simulink model "fw_safety_supervisor"  (R2026b)
settings: Solver=VariableStepAuto
undefined symbols (not defined in the file or in its folder): ImplementType, P, ShaddadMode, Ts
libraries: simulink x65
settings Model: Creator=aomar  LastModifiedBy=aomar

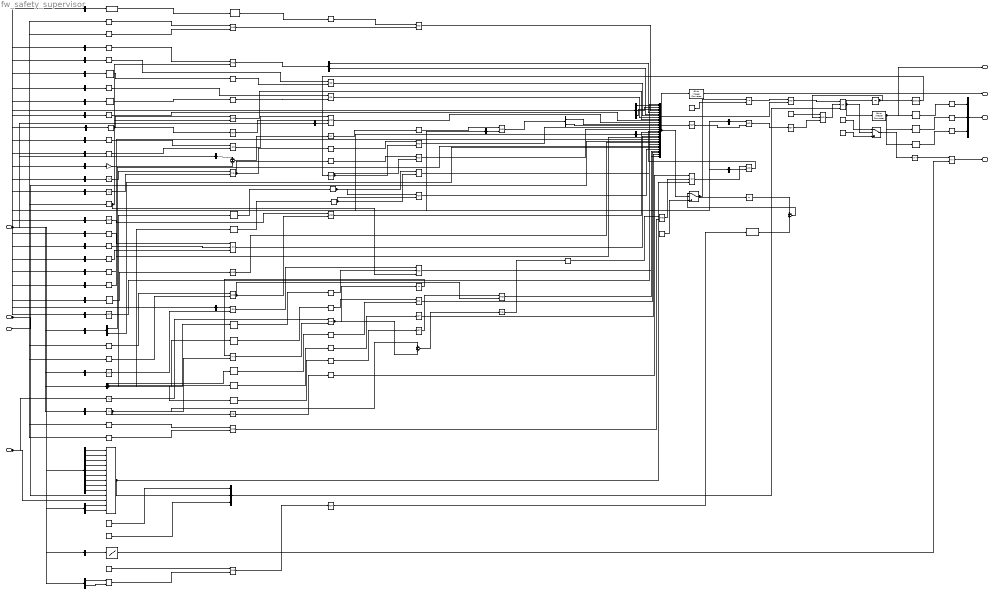
== system fw_safety_supervisor ==
  fw10 : Inport  SampleTime=Ts.ctrl
  mode_prev : Inport  Port=2  OutDataTypeStr=uint8  SampleTime=Ts.ctrl
  stop_fail_prev : Inport  Port=3  OutDataTypeStr=boolean  SampleTime=Ts.ctrl
  vtrack_ref_prev : Inport  Port=4  OutDataTypeStr=single  PortDimensions=2  SampleTime=Ts.ctrl
  Act : Logic  AllPortsSameDT=off  OutDataTypeStr=boolean
  Act_hi : simulink/Logic and Bit Operations/Compare To Constant  relop=<=  const=double(ShaddadMode.CTRL_STOP)  OutDataTypeStr=boolean
  Act_lo : simulink/Logic and Bit Operations/Compare To Constant  relop=>=  const=double(ShaddadMode.MANUAL)  OutDataTypeStr=boolean
  Active : Logic  Operator=OR  Inputs=3  AllPortsSameDT=off  OutDataTypeStr=boolean
  Auto : Logic  AllPortsSameDT=off  OutDataTypeStr=boolean
  Auto_hi : simulink/Logic and Bit Operations/Compare To Constant  relop=<=  const=double(ShaddadMode.AUTO)  OutDataTypeStr=boolean
  Auto_lo : simulink/Logic and Bit Operations/Compare To Constant  relop=>=  const=double(ShaddadMode.AUTO_START)  OutDataTypeStr=boolean
  Bms_dcl_low : simulink/Logic and Bit Operations/Compare To Constant  relop=<  const=P.electronics.safety.dcl_warn  OutDataTypeStr=boolean
  Bms_fresh : Logic  Operator=NOT  Inputs=1  AllPortsSameDT=off  OutDataTypeStr=boolean
  Bms_stale : simulink/Logic and Bit Operations/Compare To Constant  relop=>  const=P.electronics.safety.bms_timeout + Ts.hk/2  OutDataTypeStr=boolean
  Bms_warn_any : Logic  Operator=OR  AllPortsSameDT=off  OutDataTypeStr=boolean
  Bms_warnword : simulink/Logic and Bit Operations/Compare To Zero  relop=~=  OutDataTypeStr=boolean
  Busoff : Demux  Outputs=2
  C00_hw_estop : Logic  Operator=NAND  AllPortsSameDT=off  OutDataTypeStr=boolean
  C04_comp_timeout : Logic  AllPortsSameDT=off  OutDataTypeStr=boolean
  C07_drv_fault_L : Logic  Operator=OR  AllPortsSameDT=off  OutDataTypeStr=boolean
  C08_drv_fault_R : Logic  Operator=OR  AllPortsSameDT=off  OutDataTypeStr=boolean
  C09_bms_timeout : Logic  AllPortsSameDT=off  OutDataTypeStr=boolean
  C10_bms_alarm : simulink/Logic and Bit Operations/Compare To Constant  relop===  const=3  OutDataTypeStr=boolean
  C11_bms_warn : Logic  Inputs=3  AllPortsSameDT=off  OutDataTypeStr=boolean
  C14_tilt_warn : Logic  AllPortsSameDT=off  OutDataTypeStr=boolean
  C15_tilt_stop : Logic  AllPortsSameDT=off  OutDataTypeStr=boolean
  C16_overspeed : Logic  AllPortsSameDT=off  OutDataTypeStr=boolean
  C17_hv_lost : Logic  AllPortsSameDT=off  OutDataTypeStr=boolean
  C19_rail_uv : Logic  Operator=OR  Inputs=3  AllPortsSameDT=off  OutDataTypeStr=boolean
  C20_encl_warn : simulink/Logic and Bit Operations/Compare To Constant  relop=>  const=P.electronics.safety.T_encl_warn  OutDataTypeStr=boolean
  C21_encl_crit : simulink/Logic and Bit Operations/Compare To Constant  relop=>  const=P.electronics.safety.T_encl_crit  OutDataTypeStr=boolean
  C23_overrun : Logic  Inputs=1  AllPortsSameDT=off  OutDataTypeStr=boolean
  C24_imu_fault : Logic  Operator=NOT  Inputs=1  AllPortsSameDT=off  OutDataTypeStr=boolean
  C27_discrepancy : Logic  Operator=XOR  AllPortsSameDT=off  OutDataTypeStr=boolean
  C28_impl_fault : Logic  Inputs=3  AllPortsSameDT=off  OutDataTypeStr=boolean
  C29_bumper : Logic  Operator=OR  AllPortsSameDT=off  OutDataTypeStr=boolean
  C30_lid_open : Logic  Operator=NOT  Inputs=1  AllPortsSameDT=off  OutDataTypeStr=boolean
  C31_relay_open : Logic  AllPortsSameDT=off  OutDataTypeStr=boolean
  Clear : Logic  AllPortsSameDT=off  OutDataTypeStr=boolean
  Cls : Concatenate  NumInputs=3
  Cls_A : simulink/Logic and Bit Operations/Compare To Zero  relop=~=  OutDataTypeStr=boolean
  Cls_A_mask : simulink/Logic and Bit Operations/Bitwise Operator  logicop=AND  UseBitMask=on  BitMask=P.electronics.safety.maskA  BitMaskRealWorld=Stored Integer
  Cls_B : simulink/Logic and Bit Operations/Compare To Zero  relop=~=  OutDataTypeStr=boolean
  Cls_B_mask : simulink/Logic and Bit Operations/Bitwise Operator  logicop=AND  UseBitMask=on  BitMask=P.electronics.safety.maskB  BitMaskRealWorld=Stored Integer
  Cls_C : simulink/Logic and Bit Operations/Compare To Zero  relop=~=  OutDataTypeStr=boolean
  Cls_C_mask : simulink/Logic and Bit Operations/Bitwise Operator  logicop=AND  UseBitMask=on  BitMask=P.electronics.safety.maskC  BitMaskRealWorld=Stored Integer
  Cnt : Switch  Criteria=u2 ~= 0  SaturateOnIntegerOverflow=off  InputSameDT=off
  Cnt_inc : Sum  OutDataTypeStr=uint16  SaturateOnIntegerOverflow=on
  Cnt_prev : UnitDelay  InitialCondition=zeros(1,32)  SampleTime=-1
  Cnt_zero : Constant  Value=zeros(1,32)  OutDataTypeStr=uint16  SampleTime=Ts.ctrl
  Cond : Concatenate  NumInputs=32
  Cond_not : Logic  Operator=NOT  Inputs=1  AllPortsSameDT=off  OutDataTypeStr=boolean
  Count_tick : Logic  Operator=NOT  Inputs=1  AllPortsSameDT=off  OutDataTypeStr=boolean
  DI_bumper_front : simulink/Logic and Bit Operations/Compare To Zero  relop=~=  OutDataTypeStr=boolean
  DI_bumper_front_mask : simulink/Logic and Bit Operations/Bitwise Operator  logicop=AND  UseBitMask=on  BitMask=2^(P.electronics.di.bumper_front)  BitMaskRealWorld=Stored Integer
  DI_bumper_rear : simulink/Logic and Bit Operations/Compare To Zero  relop=~=  OutDataTypeStr=boolean
  DI_bumper_rear_mask : simulink/Logic and Bit Operations/Bitwise Operator  logicop=AND  UseBitMask=on  BitMask=2^(P.electronics.di.bumper_rear)  BitMaskRealWorld=Stored Integer
  DI_estop_ch1_ok : simulink/Logic and Bit Operations/Compare To Zero  relop=~=  OutDataTypeStr=boolean
  DI_estop_ch1_ok_mask : simulink/Logic and Bit Operations/Bitwise Operator  logicop=AND  UseBitMask=on  BitMask=2^(P.electronics.di.estop_ch1_ok)  BitMaskRealWorld=Stored Integer
  DI_estop_ch2_ok : simulink/Logic and Bit Operations/Compare To Zero  relop=~=  OutDataTypeStr=boolean
  DI_estop_ch2_ok_mask : simulink/Logic and Bit Operations/Bitwise Operator  logicop=AND  UseBitMask=on  BitMask=2^(P.electronics.di.estop_ch2_ok)  BitMaskRealWorld=Stored Integer
  DI_lid_closed : simulink/Logic and Bit Operations/Compare To Zero  relop=~=  OutDataTypeStr=boolean
  DI_lid_closed_mask : simulink/Logic and Bit Operations/Bitwise Operator  logicop=AND  UseBitMask=on  BitMask=2^(P.electronics.di.lid_closed)  BitMaskRealWorld=Stored Integer
  DI_safety_ok : simulink/Logic and Bit Operations/Compare To Zero  relop=~=  OutDataTypeStr=boolean
  DI_safety_ok_mask : simulink/Logic and Bit Operations/Bitwise Operator  logicop=AND  UseBitMask=on  BitMask=2^(P.electronics.di.safety_ok)  BitMaskRealWorld=Stored Integer
  Derate_bits : MinMax
  Derate_one : Constant  Value=ones(1,32)  OutDataTypeStr=single  SampleTime=Ts.ctrl
  Derate_sel : Switch  Criteria=u2 ~= 0  SaturateOnIntegerOverflow=off  InputSameDT=off
  Derate_therm : Lookup_n-D  NumberOfTableDimensions=1  BreakpointsForDimension1=P.electronics.aux.derate_bp  BreakpointsForDimension1DataTypeStr=single  Table=P.electronics.aux.derate_k  TableDataTypeStr=single  ExtrapMethod=Clip  InternalRulePriority=Speed  OutDataTypeStr=single  RndMeth=Simplest
  Derate_vec : Constant  Value=P.electronics.safety.derate_vec  OutDataTypeStr=single  SampleTime=Ts.ctrl
  Descent_trip : Subsystem
  Drv_old : simulink/Logic and Bit Operations/Compare To Constant  relop=>  const=P.electronics.safety.drv_timeout + Ts.ctrl/2  OutDataTypeStr=boolean
  Drv_on : Logic  AllPortsSameDT=off  OutDataTypeStr=boolean
  Drv_on_hi : simulink/Logic and Bit Operations/Compare To Constant  relop=<=  const=double(ShaddadMode.AUTO)  OutDataTypeStr=boolean
  Drv_on_lo : simulink/Logic and Bit Operations/Compare To Constant  relop=>=  const=double(ShaddadMode.MANUAL)  OutDataTypeStr=boolean
  Drv_tmo : Logic  AllPortsSameDT=off  OutDataTypeStr=boolean
  Drv_tmo_LR : Demux  Outputs=2
  Enc_abs : Abs  SaturateOnIntegerOverflow=off
  Enc_bad : simulink/Logic and Bit Operations/Compare To Constant  relop=>  const=P.electronics.drv.enc_mismatch_v  OutDataTypeStr=boolean
  Enc_diff : Sum  Inputs=+-
  Enc_mis : Logic  AllPortsSameDT=off  OutDataTypeStr=boolean
  Enc_mis_LR : Demux  Outputs=2
  Esc_fault_L : simulink/Logic and Bit Operations/Compare To Constant  relop===  const=P.electronics.safety.esc_fault_state  OutDataTypeStr=boolean
  Esc_fault_R : simulink/Logic and Bit Operations/Compare To Constant  relop===  const=P.electronics.safety.esc_fault_state  OutDataTypeStr=boolean
  Fault_pack : simulink/Logic and Bit Operations/Bit to Integer Converter  nbits=32  bitOrder=LSB first  signedOutputValues=Unsigned  outDtype=uint32  outDtypeSigned=Inherit via internal rule
      settings: LibrarySourceBlock=|
      | commutil2/Bit to Integer
      | Converter
  Fc_mask_L : simulink/Logic and Bit Operations/Bitwise Operator  logicop=AND  UseBitMask=on  BitMask=P.electronics.safety.drv_fault_mask  BitMaskRealWorld=Stored Integer
  Fc_mask_R : simulink/Logic and Bit Operations/Bitwise Operator  logicop=AND  UseBitMask=on  BitMask=P.electronics.safety.drv_fault_mask  BitMaskRealWorld=Stored Integer
  Fc_on_L : simulink/Logic and Bit Operations/Compare To Zero  relop=~=  OutDataTypeStr=boolean
  Fc_on_R : simulink/Logic and Bit Operations/Compare To Zero  relop=~=  OutDataTypeStr=boolean
  Follow_err : Sum  Inputs=+-
  Follow_max : MinMax  Function=max
  Follow_on : Logic  AllPortsSameDT=off  OutDataTypeStr=boolean
  Follow_over : simulink/Logic and Bit Operations/Compare To Constant  relop=>  const=P.electronics.lim.v_follow_dv  OutDataTypeStr=boolean
  Gate_bits : Constant  Value=bitget(sum(2.^[14 15]), 1:32) ~= 0  OutDataTypeStr=boolean  SampleTime=Ts.ctrl
  Gate_closed : Logic  Operator=NAND  AllPortsSameDT=off  OutDataTypeStr=boolean
  Held : Logic  Inputs=3  AllPortsSameDT=off  OutDataTypeStr=boolean
  Hold_tick : Logic  AllPortsSameDT=off  OutDataTypeStr=boolean
  Hv_not_ready : Logic  Operator=NOT  Inputs=1  AllPortsSameDT=off  OutDataTypeStr=boolean
  Imm : Concatenate  NumInputs=3
  Imm_hi : Constant  Value=false(1,15)  OutDataTypeStr=boolean  SampleTime=Ts.ctrl
  Imm_lo : Constant  Value=false(1,16)  OutDataTypeStr=boolean  SampleTime=Ts.ctrl
  Impl_bad : Logic  Operator=OR  AllPortsSameDT=off  OutDataTypeStr=boolean
  Impl_fitted : simulink/Logic and Bit Operations/Compare To Zero  relop=~=  OutDataTypeStr=boolean
  Impl_id_mask : simulink/Logic and Bit Operations/Bitwise Operator  logicop=AND  UseBitMask=on  BitMask=2^P.electronics.di.impl_id0 + 2^P.electronics.di.impl_id1  BitMaskRealWorld=Stored Integer
  Impl_no_rx : Logic  Operator=NOT  Inputs=1  AllPortsSameDT=off  OutDataTypeStr=boolean
  Imu_fault_prev : Selector  InputPortWidth=32  IndexOptions=Index vector (dialog)  Indices=1 + 24  OutputSizes=1
  Imu_ok_prev : Logic  Operator=NOT  Inputs=1  AllPortsSameDT=off  OutDataTypeStr=boolean
  Inc : DataTypeConversion  OutDataTypeStr=uint16  RndMeth=Round
  K_der_min : MinMax  Inputs=2
  Keep : Logic  Operator=NOT  Inputs=1  AllPortsSameDT=off  OutDataTypeStr=boolean
  Latch_mask : Constant  Value=bitget(double(P.electronics.safety.latch_mask), 1:32) ~= 0  OutDataTypeStr=boolean  SampleTime=Ts.ctrl
  Mon : simulink/Logic and Bit Operations/Compare To Constant  relop=>=  const=double(ShaddadMode.STANDBY)  OutDataTypeStr=boolean
  N_persist : Constant  Value=round(P.electronics.safety.t_persist/Ts.ctrl) + 1  OutDataTypeStr=uint16  SampleTime=Ts.ctrl
  Over_any : Logic  Operator=OR  Inputs=3  AllPortsSameDT=off  OutDataTypeStr=boolean
  Ovr_taps : simulink/Discrete/Tapped Delay  vinit=0  samptime=-1  NumDelays=P.electronics.safety.overrun_n - 1  DelayOrder=Oldest  includeCurrent=on
  Persisted : Logic  AllPortsSameDT=off  OutDataTypeStr=boolean
  Persisted_t : RelationalOperator  OutDataTypeStr=boolean  RndMeth=Simplest  InputSameDT=off
  Pitch_abs : Abs  SaturateOnIntegerOverflow=off
  Q_prev : UnitDelay  InitialCondition=false(1,32)  SampleTime=-1
  Relay_open : Logic  Operator=NOT  Inputs=1  AllPortsSameDT=off  OutDataTypeStr=boolean
  Rf : MinMax  Function=max  Inputs=2
  Rf_low : MinMax  Inputs=2
  Rf_prev : UnitDelay  InitialCondition=[0 0]  SampleTime=-1
  Roll_abs : Abs  SaturateOnIntegerOverflow=off
  Sel_DCL : BusSelector  OutputSignals=bms.DCL
  Sel_T_encl_crit : BusSelector  OutputSignals=adc.T_encl
  Sel_T_encl_derate : BusSelector  OutputSignals=adc.T_encl
  Sel_T_encl_warn : BusSelector  OutputSignals=adc.T_encl
  Sel_V12 : BusSelector  OutputSignals=adc.V12
  Sel_V24 : BusSelector  OutputSignals=adc.V24
  Sel_V5 : BusSelector  OutputSignals=adc.V5
  Sel_bms_age : BusSelector  OutputSignals=bms_age
  Sel_bms_valid : BusSelector  OutputSignals=bms.valid
  Sel_brake_rel : BusSelector  OutputSignals=drive_fb.L.brake_released,drive_fb.R.brake_released
  Sel_busoff : BusSelector  OutputSignals=busoff
  Sel_descent : BusSelector  OutputSignals=tilt.pitch,tilt.imu_valid,di_word,impl.impl_type,impl.rx_ok,adc.lift_pos,odom.vTrack_LR,a_track,odom.valid
  Sel_di_word : BusSelector  OutputSignals=di_word
  Sel_drv_age : BusSelector  OutputSignals=drv_age
  Sel_fault_code_L : BusSelector  OutputSignals=drive_fb.L.fault_code
  Sel_fault_code_R : BusSelector  OutputSignals=drive_fb.R.fault_code
  Sel_fault_level : BusSelector  OutputSignals=bms.fault_level
  Sel_hv_opening : BusSelector  OutputSignals=bms.hv_opening_warn
  Sel_hv_ready : BusSelector  OutputSignals=bms.hv_ready
  Sel_impl_fault : BusSelector  OutputSignals=impl.fault
  Sel_imu_valid_fault : BusSelector  OutputSignals=tilt.imu_valid
  Sel_odom_valid_enc : BusSelector  OutputSignals=odom.valid
  Sel_odom_valid_over : BusSelector  OutputSignals=odom.valid
  Sel_overrun : BusSelector  OutputSignals=overrun
  Sel_pitch : BusSelector  OutputSignals=tilt.pitch
  Sel_rc : BusSelector  OutputSignals=rc.estop_remote,rc.rc_link_lost,rc.failsafe
  Sel_reset_req : BusSelector  OutputSignals=reset_req
  Sel_roll : BusSelector  OutputSignals=tilt.roll
  Sel_rx_ok : BusSelector  OutputSignals=impl.rx_ok
  Sel_seq : BusSelector  OutputSignals=gnc_cmd.seq
  Sel_state_L : BusSelector  OutputSignals=drive_fb.L.state
  Sel_state_R : BusSelector  OutputSignals=drive_fb.R.state
  Sel_tilt_gate : BusSelector  OutputSignals=tilt.tilt_gate,tilt.imu_valid
  Sel_vTrack_enc : BusSelector  OutputSignals=odom.vTrack_LR
  Sel_vTrack_over : BusSelector  OutputSignals=odom.vTrack_LR
  Sel_wMotor_LR : BusSelector  OutputSignals=odom.wMotor_LR
  Sel_warn_word : BusSelector  OutputSignals=bms.warn_word
  Seq_age : Subsystem
  Seq_change : simulink/Logic and Bit Operations/Detect Change  vinit=0  OutDataTypeStr=boolean
  Seq_stale : simulink/Logic and Bit Operations/Compare To Constant  relop=>=  const=round(P.electronics.safety.comp_timeout/Ts.ctrl)  OutDataTypeStr=boolean
  Tilt_gt_stop : simulink/Logic and Bit Operations/Compare To Constant  relop=>  const=P.electronics.safety.tilt_stop  OutDataTypeStr=boolean
  Tilt_gt_warn : simulink/Logic and Bit Operations/Compare To Constant  relop=>  const=P.electronics.safety.tilt_warn  OutDataTypeStr=boolean
  Tilt_max : MinMax  Function=max  Inputs=2
  V12_low : simulink/Logic and Bit Operations/Compare To Constant  relop=<  const=P.electronics.safety.V12_min  OutDataTypeStr=boolean
  V24_low : simulink/Logic and Bit Operations/Compare To Constant  relop=<  const=P.electronics.safety.V24_min  OutDataTypeStr=boolean
  V5_low : simulink/Logic and Bit Operations/Compare To Constant  relop=<  const=P.electronics.safety.V5_min  OutDataTypeStr=boolean
  Vref_abs : Abs  SaturateOnIntegerOverflow=off
  Vt_abs : Abs  SaturateOnIntegerOverflow=off
  Vt_max : MinMax  Function=max
  Vt_over : simulink/Logic and Bit Operations/Compare To Constant  relop=>  const=P.electronics.lim.v_overspeed  OutDataTypeStr=boolean
  Warn_pack : simulink/Logic and Bit Operations/Bit to Integer Converter  nbits=32  bitOrder=LSB first  signedOutputValues=Unsigned  outDtype=uint32  outDtypeSigned=Inherit via internal rule
      settings: LibrarySourceBlock=|
      | commutil2/Bit to Integer
      | Converter
  Wm_to_v : Gain  Gain=1/P.electronics.drv.k_v2w
  fault_word : Outport  OutDataTypeStr=uint32
  warn_word : Outport  Port=2  OutDataTypeStr=uint32
  fault_cls : Outport  Port=3  OutDataTypeStr=boolean
  k_der : Outport  Port=4  OutDataTypeStr=single
  wires:
  fw10/1 -> Sel_tilt_gate/1, Sel_T_encl_derate/1, Sel_brake_rel/1, Sel_descent/1, Sel_seq/1, Sel_vTrack_over/1, Sel_drv_age/1, Sel_state_L/1, Sel_di_word/1, Sel_fault_code_L/1, Sel_rx_ok/1, Sel_state_R/1, Sel_fault_code_R/1, Sel_rc/1, Sel_fault_level/1, Sel_reset_req/1, Sel_busoff/1, Sel_bms_valid/1, Sel_bms_age/1, Sel_odom_valid_enc/1, Sel_hv_opening/1, Sel_imu_valid_fault/1, Sel_warn_word/1, Sel_impl_fault/1, Sel_DCL/1, Sel_overrun/1, Sel_vTrack_enc/1, Sel_wMotor_LR/1, Sel_T_encl_crit/1, Sel_odom_valid_over/1, Sel_roll/1, Sel_T_encl_warn/1, Sel_pitch/1, Sel_V5/1, Sel_V12/1, Sel_hv_ready/1, Sel_V24/1  "fw10"
  mode_prev/1 -> Auto_lo/1, Auto_hi/1, Descent_trip/10(mode_prev), Drv_on_hi/1, Mon/1, Drv_on_lo/1, Act_hi/1, Act_lo/1  "mode_prev"
  stop_fail_prev/1 -> Cond/23  "stop_fail_prev"
  vtrack_ref_prev/1 -> Vref_abs/1, Descent_trip/11(vref_LR)  "vtrack_ref_prev"
  Sel_seq/1 -> Seq_change/1  "<seq>"
  Sel_drv_age/1 -> Drv_old/1  "<drv_age>"
  Sel_state_L/1 -> Esc_fault_L/1  "<state>"
  Sel_fault_code_L/1 -> Fc_mask_L/1  "<fault_code>"
  Sel_state_R/1 -> Esc_fault_R/1  "<state>"
  Sel_fault_code_R/1 -> Fc_mask_R/1  "<fault_code>"
  Sel_fault_level/1 -> C10_bms_alarm/1  "<fault_level>"
  Sel_warn_word/1 -> Bms_warnword/1  "<warn_word>"
  Sel_DCL/1 -> Bms_dcl_low/1  "<DCL>"
  Sel_wMotor_LR/1 -> Wm_to_v/1  "<wMotor_LR>"
  Sel_roll/1 -> Roll_abs/1  "<roll>"
  Sel_pitch/1 -> Pitch_abs/1  "<pitch>"
  Sel_hv_ready/1 -> Hv_not_ready/1  "<hv_ready>"
  Sel_V24/1 -> V24_low/1  "<V24>"
  Sel_V12/1 -> V12_low/1  "<V12>"
  Sel_V5/1 -> V5_low/1  "<V5>"
  Sel_T_encl_warn/1 -> C20_encl_warn/1  "<T_encl>"
  Sel_T_encl_crit/1 -> C21_encl_crit/1  "<T_encl>"
  Sel_overrun/1 -> Ovr_taps/1  "<overrun>"
  Sel_imu_valid_fault/1 -> C24_imu_fault/1  "<imu_valid>"
  Sel_busoff/1 -> Busoff/1  "<busoff>"
  Sel_rx_ok/1 -> Impl_no_rx/1  "<rx_ok>"
  Sel_vTrack_over/1 -> Vt_abs/1  "<vTrack_LR>"
  Sel_descent/1 -> Descent_trip/1(pitch)  "<pitch>"
  Sel_descent/2 -> Descent_trip/2(imu_valid)  "<imu_valid>"
  Sel_descent/3 -> Descent_trip/3(di_word)  "<di_word>"
  Sel_descent/4 -> Descent_trip/4(impl_type)  "<impl_type>"
  Sel_descent/5 -> Descent_trip/5(impl_rx_ok)  "<rx_ok>"
  Sel_descent/6 -> Descent_trip/6(lift_pos)  "<lift_pos>"
  Sel_descent/7 -> Descent_trip/7(v_LR)  "<vTrack_LR>"
  Sel_descent/8 -> Descent_trip/8(a_track)  "<a_track>"
  Sel_descent/9 -> Descent_trip/9(odom_valid)  "<valid>"
  Sel_brake_rel/1 -> Descent_trip/12(brake_rel_L)  "<brake_released>"
  Sel_brake_rel/2 -> Descent_trip/13(brake_rel_R)  "<brake_released>"
  Sel_T_encl_derate/1 -> Derate_therm/1  "<T_encl>"
  Sel_tilt_gate/1 -> Gate_closed/1  "<tilt_gate>"
  Sel_tilt_gate/2 -> Gate_closed/2  "<imu_valid>"
  Sel_bms_age/1 -> Bms_stale/1  "<bms_age>"
  Busoff/1 -> Cond/26  "can1_busoff"
  Busoff/2 -> Cond/27  "can2_busoff"
  Sel_di_word/1 -> DI_estop_ch1_ok_mask/1, DI_estop_ch2_ok_mask/1, Impl_id_mask/1, DI_bumper_front_mask/1, DI_bumper_rear_mask/1, DI_safety_ok_mask/1, DI_lid_closed_mask/1  "<di_word>"
  Auto_lo/1 -> Auto/1  "Auto_lo"
  Auto_hi/1 -> Auto/2  "Auto_hi"
  Drv_old/1 -> Drv_tmo/1  "Drv_old"
  Esc_fault_L/1 -> C07_drv_fault_L/1  "Esc_fault_L"
  Esc_fault_R/1 -> C08_drv_fault_R/1  "Esc_fault_R"
  C10_bms_alarm/1 -> Cond/11  "C10_bms_alarm"
  Bms_warnword/1 -> Bms_warn_any/1  "Bms_warnword"
  Bms_dcl_low/1 -> Bms_warn_any/2  "Bms_dcl_low"
  Wm_to_v/1 -> Enc_diff/2  "Wm_to_v"
  Roll_abs/1 -> Tilt_max/1  "Roll_abs"
  Pitch_abs/1 -> Tilt_max/2  "Pitch_abs"
  Mon/1 -> Drv_tmo/2, C09_bms_timeout/2, C28_impl_fault/3  "Mon"
  Hv_not_ready/1 -> C17_hv_lost/1  "Hv_not_ready"
  V24_low/1 -> C19_rail_uv/1  "V24_low"
  V12_low/1 -> C19_rail_uv/2  "V12_low"
  V5_low/1 -> C19_rail_uv/3  "V5_low"
  C20_encl_warn/1 -> Cond/21  "C20_encl_warn"
  C21_encl_crit/1 -> Cond/22  "C21_encl_crit"
  C24_imu_fault/1 -> Cond/25  "C24_imu_fault"
  Act_lo/1 -> Act/1  "Act_lo"
  Act_hi/1 -> Act/2  "Act_hi"
  Impl_no_rx/1 -> Impl_bad/2  "Impl_no_rx"
  Vref_abs/1 -> Rf/1  "vtrack_ref_abs"
  Vt_abs/1 -> Follow_err/1, Rf_low/2, Vt_max/1  "Vt_abs"
  Drv_on_lo/1 -> Drv_on/1  "Drv_on_lo"
  Drv_on_hi/1 -> Drv_on/2  "Drv_on_hi"
  Imm_lo/1 -> Imm/1  "Imm_lo"
  Imm_hi/1 -> Imm/3  "Imm_hi"
  Gate_bits/1 -> Hold_tick/1  "Gate_bits"
  Gate_closed/1 -> Hold_tick/2  "Gate_closed"
  Ovr_taps/1 -> C23_overrun/1  "overrun_taps"
  Fc_mask_L/1 -> Fc_on_L/1  "Fc_mask_L"
  Fc_mask_R/1 -> Fc_on_R/1  "Fc_mask_R"
  Bms_stale/1 -> C09_bms_timeout/1, Bms_fresh/1  "Bms_stale"
  Descent_trip/1(cap_trip) -> Over_any/3, Imm/2  "cap_trip"
  Seq_change/1 -> Seq_age/1(fresh)  "seq_change"
  Derate_therm/1 -> K_der_min/2  "Derate_therm"
  Sel_vTrack_enc/1 -> Enc_diff/1  "<vTrack_LR>"
  Sel_impl_fault/1 -> Impl_bad/1  "<fault>"
  Imm/1 -> Active/3  "imm"
  Enc_diff/1 -> Enc_abs/1  "Enc_diff"
  Auto/1 -> C04_comp_timeout/2  "Auto"
  Drv_tmo/1 -> Drv_tmo_LR/1  "Drv_tmo"
  Fc_on_L/1 -> C07_drv_fault_L/2  "Fc_on_L"
  Fc_on_R/1 -> C08_drv_fault_R/2  "Fc_on_R"
  C09_bms_timeout/1 -> Cond/10  "C09_bms_timeout"
  Bms_fresh/1 -> C11_bms_warn/2  "Bms_fresh"
  Bms_warn_any/1 -> C11_bms_warn/1  "Bms_warn_any"
  Tilt_max/1 -> Tilt_gt_warn/1, Tilt_gt_stop/1  "tilt"
  C19_rail_uv/1 -> Cond/20  "C19_rail_uv"
  C23_overrun/1 -> Cond/24  "C23_overrun"
  Act/1 -> C17_hv_lost/2, C31_relay_open/2  "Act"
  Impl_bad/1 -> C28_impl_fault/1  "Impl_bad"
  Rf_low/1 -> Rf/2  "rf_low"
  Vt_max/1 -> Vt_over/1  "Vt_max"
  Drv_on/1 -> Follow_on/2  "drv_on"
  Hold_tick/1 -> Count_tick/1  "Hold_tick"
  DI_estop_ch1_ok_mask/1 -> DI_estop_ch1_ok/1  "DI_estop_ch1_ok_mask"
  DI_estop_ch2_ok_mask/1 -> DI_estop_ch2_ok/1  "DI_estop_ch2_ok_mask"
  Impl_id_mask/1 -> Impl_fitted/1  "Impl_id_mask"
  DI_bumper_front_mask/1 -> DI_bumper_front/1  "DI_bumper_front_mask"
  DI_bumper_rear_mask/1 -> DI_bumper_rear/1  "DI_bumper_rear_mask"
  DI_lid_closed_mask/1 -> DI_lid_closed/1  "DI_lid_closed_mask"
  DI_safety_ok_mask/1 -> DI_safety_ok/1  "DI_safety_ok_mask"
  Seq_age/1(ticks) -> Seq_stale/1  "seq_age"
  Sel_bms_valid/1 -> C11_bms_warn/3  "<valid>"
  Drv_tmo_LR/1 -> Cond/6  "drv_tmo_L"
  Drv_tmo_LR/2 -> Cond/7  "drv_tmo_R"
  Seq_stale/1 -> C04_comp_timeout/1  "Seq_stale"
  C08_drv_fault_R/1 -> Cond/9  "C08_drv_fault_R"
  C11_bms_warn/1 -> Cond/12  "C11_bms_warn"
  Enc_abs/1 -> Enc_bad/1  "Enc_abs"
  Tilt_gt_warn/1 -> C14_tilt_warn/1  "Tilt_gt_warn"
  Tilt_gt_stop/1 -> C15_tilt_stop/1  "Tilt_gt_stop"
  Imu_ok_prev/1 -> C14_tilt_warn/2, C15_tilt_stop/2  "imu_ok_prev"
  C17_hv_lost/1 -> Cond/18  "C17_hv_lost"
  Impl_fitted/1 -> C28_impl_fault/2  "Impl_fitted"
  DI_bumper_front/1 -> C29_bumper/1  "DI_bumper_front"
  Rf/1 -> Rf_prev/1, Follow_err/2  "rf"
  DI_bumper_rear/1 -> C29_bumper/2  "DI_bumper_rear"
  DI_lid_closed/1 -> C30_lid_open/1  "DI_lid_closed"
  DI_safety_ok/1 -> Relay_open/1  "DI_safety_ok"
  Vt_over/1 -> Over_any/1  "Vt_over"
  Count_tick/1 -> Inc/1  "inc"
  DI_estop_ch1_ok/1 -> C00_hw_estop/1, C27_discrepancy/1  "DI_estop_ch1_ok"
  DI_estop_ch2_ok/1 -> C00_hw_estop/2, C27_discrepancy/2  "DI_estop_ch2_ok"
  Follow_err/1 -> Follow_max/1  "follow_err_LR"
  C04_comp_timeout/1 -> Cond/5  "C04_comp_timeout"
  Enc_bad/1 -> Enc_mis/1  "Enc_bad"
  C14_tilt_warn/1 -> Cond/15  "C14_tilt_warn"
  C15_tilt_stop/1 -> Cond/16  "C15_tilt_stop"
  C00_hw_estop/1 -> Cond/1  "C00_hw_estop"
  C27_discrepancy/1 -> Cond/28  "C27_discrepancy"
  C28_impl_fault/1 -> Cond/29  "C28_impl_fault"
  C29_bumper/1 -> Cond/30  "C29_bumper"
  C30_lid_open/1 -> Cond/31  "C30_lid_open"
  Relay_open/1 -> C31_relay_open/1  "Relay_open"
  Rf_prev/1 -> Rf_low/1  "rf_prev"
  Sel_odom_valid_enc/1 -> Enc_mis/2  "<valid>"
  Enc_mis/1 -> Enc_mis_LR/1  "Enc_mis"
  C31_relay_open/1 -> Cond/32  "C31_relay_open"
  Follow_max/1 -> Follow_over/1  "follow_err"
  Enc_mis_LR/1 -> Cond/13  "enc_mis_L"
  Enc_mis_LR/2 -> Cond/14  "enc_mis_R"
  Follow_over/1 -> Follow_on/1  "Follow_over"
  Sel_rc/1 -> Cond/2  "<estop_remote>"
  Sel_rc/2 -> Cond/3  "<rc_link_lost>"
  Sel_hv_opening/1 -> Cond/19  "<hv_opening_warn>"
  Cond/1 -> Cnt/2, Warn_pack/1, Persisted/2, Cond_not/1  "cond"
  Follow_on/1 -> Over_any/2  "follow_on"
  Cnt_zero/1 -> Cnt/3  "Cnt_zero"
  N_persist/1 -> Persisted_t/2  "N_persist"
  Cond_not/1 -> Clear/2  "Cond_not"
  Over_any/1 -> C16_overspeed/1  "Over_any"
  Cnt/1 -> Persisted_t/1, Cnt_prev/1  "cnt"
  Warn_pack/1 -> warn_word/1  "warn_word"
  Sel_reset_req/1 -> Clear/1  "<reset_req>"
  Sel_odom_valid_over/1 -> C16_overspeed/2  "<valid>"
  Persisted_t/1 -> Persisted/1  "Persisted_t"
  Clear/1 -> Keep/1  "Clear"
  C16_overspeed/1 -> Cond/17  "C16_overspeed"
  Cnt_prev/1 -> Cnt_inc/1  "cnt_prev"
  Inc/1 -> Cnt_inc/2  "Inc"
  Cnt_inc/1 -> Cnt/1  "Cnt_inc"
  Persisted/1 -> Active/1  "persisted"
  Latch_mask/1 -> Held/1  "Latch_mask"
  Keep/1 -> Held/3  "Keep"
  Held/1 -> Active/2  "Held"
  Active/1 -> Derate_sel/2, Fault_pack/1, Q_prev/1  "active"
  Derate_vec/1 -> Derate_sel/1  "Derate_vec"
  Derate_one/1 -> Derate_sel/3  "Derate_one"
  Q_prev/1 -> Held/2, Imu_fault_prev/1  "q_prev"
  Derate_sel/1 -> Derate_bits/1  "Derate_sel"
  Fault_pack/1 -> fault_word/1, Cls_C_mask/1, Cls_B_mask/1, Cls_A_mask/1  "fault_word"
  Derate_bits/1 -> K_der_min/1  "Derate_bits"
  Imu_fault_prev/1 -> Imu_ok_prev/1  "imu_fault_prev"
  Cls_A_mask/1 -> Cls_A/1  "Cls_A_mask"
  Cls_B_mask/1 -> Cls_B/1  "Cls_B_mask"
  Cls_C_mask/1 -> Cls_C/1  "Cls_C_mask"
  Cls_A/1 -> Cls/1  "Cls_A"
  Cls_B/1 -> Cls/2  "Cls_B"
  Cls_C/1 -> Cls/3  "Cls_C"
  K_der_min/1 -> k_der/1  "k_der"
  Cls/1 -> fault_cls/1  "fault_cls"
  C07_drv_fault_L/1 -> Cond/8  "C07_drv_fault_L"
  Sel_rc/3 -> Cond/4  "<failsafe>"

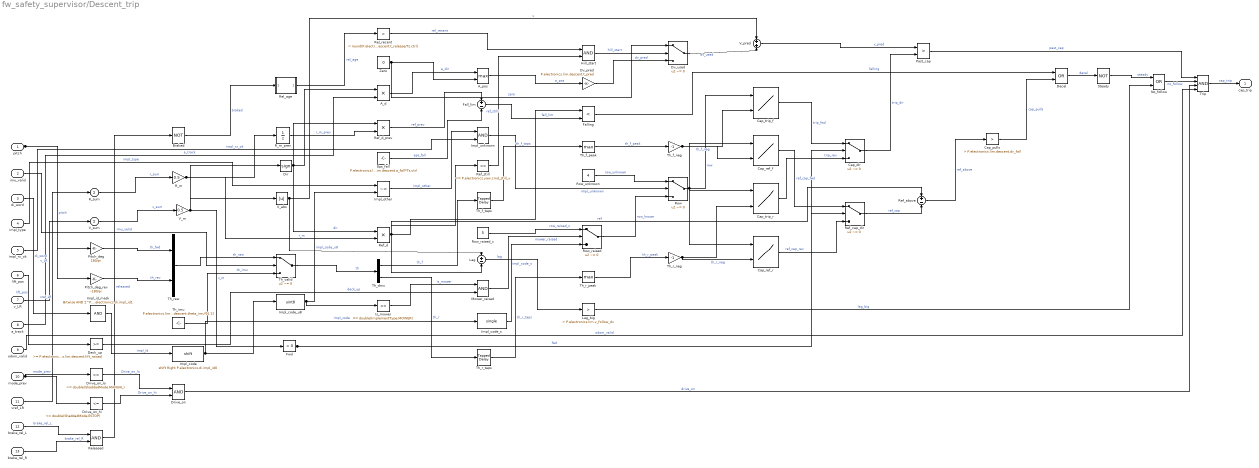
== system fw_safety_supervisor/Descent_trip ==
  pitch : Inport
  imu_valid : Inport  Port=2
  di_word : Inport  Port=3
  impl_type : Inport  Port=4
  impl_rx_ok : Inport  Port=5
  lift_pos : Inport  Port=6
  v_LR : Inport  Port=7
  a_track : Inport  Port=8
  odom_valid : Inport  Port=9
  mode_prev : Inport  Port=10
  vref_LR : Inport  Port=11
  brake_rel_L : Inport  Port=12
  brake_rel_R : Inport  Port=13
  A_d : Product  Inputs=**
  A_pos : MinMax  Function=max  Inputs=2
  Braked : Logic  Operator=NOT  Inputs=1  AllPortsSameDT=off  OutDataTypeStr=boolean
  Cap_dir : Switch  Criteria=u2 ~= 0  SaturateOnIntegerOverflow=off  InputSameDT=off
  Cap_pulls : simulink/Logic and Bit Operations/Compare To Constant  relop=>  const=P.electronics.lim.descent.dv_fall  OutDataTypeStr=boolean
  Cap_ref_f : Lookup_n-D  BreakpointsForDimension1=0:5  BreakpointsForDimension2=-fliplr(P.electronics.lim.descent.theta_bp)  BreakpointsForDimension1DataTypeStr=single  BreakpointsForDimension2DataTypeStr=single  Table=P.electronics.lim.descent.ref_fwd(:, end:-1:1)  TableDataTypeStr=single  InterpMethod=Flat  ExtrapMethod=Clip  InternalRulePriority=Speed  OutDataTypeStr=single  RndMeth=Simplest
      settings: InputPortMap=u0,u1
  Cap_ref_r : Lookup_n-D  BreakpointsForDimension1=0:5  BreakpointsForDimension2=-fliplr(P.electronics.lim.descent.theta_bp)  BreakpointsForDimension1DataTypeStr=single  BreakpointsForDimension2DataTypeStr=single  Table=P.electronics.lim.descent.ref_rev(:, end:-1:1)  TableDataTypeStr=single  InterpMethod=Flat  ExtrapMethod=Clip  InternalRulePriority=Speed  OutDataTypeStr=single  RndMeth=Simplest
      settings: InputPortMap=u0,u1
  Cap_trip_f : Lookup_n-D  BreakpointsForDimension1=0:5  BreakpointsForDimension2=-fliplr(P.electronics.lim.descent.theta_bp)  BreakpointsForDimension1DataTypeStr=single  BreakpointsForDimension2DataTypeStr=single  Table=P.electronics.lim.descent.trip_fwd(:, end:-1:1)  TableDataTypeStr=single  InterpMethod=Flat  ExtrapMethod=Clip  InternalRulePriority=Speed  OutDataTypeStr=single  RndMeth=Simplest
      settings: InputPortMap=u0,u1
  Cap_trip_r : Lookup_n-D  BreakpointsForDimension1=0:5  BreakpointsForDimension2=-fliplr(P.electronics.lim.descent.theta_bp)  BreakpointsForDimension1DataTypeStr=single  BreakpointsForDimension2DataTypeStr=single  Table=P.electronics.lim.descent.trip_rev(:, end:-1:1)  TableDataTypeStr=single  InterpMethod=Flat  ExtrapMethod=Clip  InternalRulePriority=Speed  OutDataTypeStr=single  RndMeth=Simplest
      settings: InputPortMap=u0,u1
  Decel : Logic  Operator=OR  AllPortsSameDT=off  OutDataTypeStr=boolean
  Deck_up : simulink/Logic and Bit Operations/Compare To Constant  relop=>=  const=P.electronics.lim.descent.lift_raised  OutDataTypeStr=boolean
  Dir : Signum
  Drive_on : Logic  AllPortsSameDT=off  OutDataTypeStr=boolean
  Drive_on_hi : simulink/Logic and Bit Operations/Compare To Constant  relop=<=  const=double(ShaddadMode.ESTOP)  OutDataTypeStr=boolean
  Drive_on_lo : simulink/Logic and Bit Operations/Compare To Constant  relop=>=  const=double(ShaddadMode.MANUAL)  OutDataTypeStr=boolean
  Dv_pred : Gain  Gain=P.electronics.lim.descent.t_pred
  Dv_used : Switch  Criteria=u2 ~= 0  SaturateOnIntegerOverflow=off  InputSameDT=off
  Eps_fall : Constant  Value=P.electronics.lim.descent.a_fall*Ts.ctrl  OutDataTypeStr=single  SampleTime=Ts.ctrl
  Fall_lim : Sum  Inputs=+-
  Falling : RelationalOperator  Operator=<  OutDataTypeStr=boolean  RndMeth=Simplest  InputSameDT=off
  Fwd : simulink/Logic and Bit Operations/Compare To Zero  relop=>  OutDataTypeStr=boolean
  Hill_start : Logic  AllPortsSameDT=off  OutDataTypeStr=boolean
  Impl_code : ArithShift  BitShiftNumber=P.electronics.di.impl_id0  BitShiftDirection=Right
  Impl_code_s : DataTypeConversion  OutDataTypeStr=single  RndMeth=Round
  Impl_code_u8 : DataTypeConversion  OutDataTypeStr=uint8  RndMeth=Round
  Impl_id_mask : simulink/Logic and Bit Operations/Bitwise Operator  logicop=AND  UseBitMask=on  BitMask=2^P.electronics.di.impl_id0 + 2^P.electronics.di.impl_id1  BitMaskRealWorld=Stored Integer
  Impl_other : RelationalOperator  Operator=~=  OutDataTypeStr=boolean  RndMeth=Simplest  InputSameDT=off
  Impl_unknown : Logic  AllPortsSameDT=off  OutDataTypeStr=boolean
  Is_mower : simulink/Logic and Bit Operations/Compare To Constant  relop===  const=double(ImplementType.MOWER)  OutDataTypeStr=boolean
  Lag : Sum  Inputs=+-
  Lag_big : simulink/Logic and Bit Operations/Compare To Constant  relop=>  const=P.electronics.lim.v_follow_dv  OutDataTypeStr=boolean
  Mower_raised : Logic  AllPortsSameDT=off  OutDataTypeStr=boolean
  No_follow : Logic  Operator=OR  AllPortsSameDT=off  OutDataTypeStr=boolean
  Past_cap : RelationalOperator  Operator=>  OutDataTypeStr=boolean  RndMeth=Simplest  InputSameDT=off
  Pitch_deg : Gain  Gain=180/pi
  Pitch_deg_rev : Gain  Gain=-180/pi
  R_m : Gain  Gain=0.5
  R_m_prev : UnitDelay  SampleTime=-1
  R_sum : Sum  Inputs=+
  Ref_above : Sum  Inputs=+-
  Ref_cap_dir : Switch  Criteria=u2 ~= 0  SaturateOnIntegerOverflow=off  InputSameDT=off
  Ref_d : Product  Inputs=**
  Ref_d_prev : Product  Inputs=**
  Ref_still : simulink/Logic and Bit Operations/Compare To Constant  relop=<=  const=P.electronics.yaw.cmd_still_v  OutDataTypeStr=boolean
  Rel_age : Subsystem
  Rel_recent : simulink/Logic and Bit Operations/Compare To Constant  relop=<  const=round(P.electronics.lim.descent.t_release/Ts.ctrl)  OutDataTypeStr=boolean
  Released : Logic  AllPortsSameDT=off  OutDataTypeStr=boolean
  Row : Switch  Criteria=u2 ~= 0  SaturateOnIntegerOverflow=off  InputSameDT=off
  Row_raised : Switch  Criteria=u2 ~= 0  SaturateOnIntegerOverflow=off  InputSameDT=off
  Row_raised_c : Constant  Value=5  OutDataTypeStr=single  SampleTime=Ts.ctrl
  Row_unknown : Constant  Value=4  OutDataTypeStr=single  SampleTime=Ts.ctrl
  Steady : Logic  Operator=NOT  Inputs=1  AllPortsSameDT=off  OutDataTypeStr=boolean
  Th_dmx : Demux  Outputs=2
  Th_f_neg : Gain  Gain=-1
  Th_f_peak : MinMax  Function=max
  Th_f_taps : simulink/Discrete/Tapped Delay  vinit=P.electronics.lim.descent.theta_imu  samptime=-1  NumDelays=round(P.electronics.lim.descent.t_hold/Ts.ctrl) - 1  DelayOrder=Oldest  includeCurrent=on
  Th_imu : Constant  Value=P.electronics.lim.descent.theta_imu*[1 1]  OutDataTypeStr=single  SampleTime=Ts.ctrl
  Th_r_neg : Gain  Gain=-1
  Th_r_peak : MinMax  Function=max
  Th_r_taps : simulink/Discrete/Tapped Delay  vinit=P.electronics.lim.descent.theta_imu  samptime=-1  NumDelays=round(P.electronics.lim.descent.t_hold/Ts.ctrl) - 1  DelayOrder=Oldest  includeCurrent=on
  Th_raw : Concatenate
  Th_valid : Switch  Criteria=u2 ~= 0  SaturateOnIntegerOverflow=off  InputSameDT=off
  Trip : Logic  Inputs=4  AllPortsSameDT=off  OutDataTypeStr=boolean
  V_abs : Abs  SaturateOnIntegerOverflow=off
  V_m : Gain  Gain=0.5
  V_pred : Sum
  V_sum : Sum  Inputs=+
  Zero : Constant  Value=0  OutDataTypeStr=single  SampleTime=Ts.ctrl
  cap_trip : Outport
  wires:
  pitch/1 -> Pitch_deg_rev/1, Pitch_deg/1  "pitch"
  imu_valid/1 -> Th_valid/2  "imu_valid"
  di_word/1 -> Impl_id_mask/1  "di_word"
  impl_type/1 -> Impl_other/1  "impl_type"
  impl_rx_ok/1 -> Impl_unknown/2  "impl_rx_ok"
  lift_pos/1 -> Deck_up/1  "lift_pos"
  v_LR/1 -> V_sum/1  "v_LR"
  a_track/1 -> A_d/2  "a_track"
  odom_valid/1 -> Trip/4  "odom_valid"
  mode_prev/1 -> Drive_on_hi/1, Drive_on_lo/1  "mode_prev"
  vref_LR/1 -> R_sum/1  "vref_LR"
  brake_rel_L/1 -> Released/1  "brake_rel_L"
  brake_rel_R/1 -> Released/2  "brake_rel_R"
  R_sum/1 -> R_m/1  "r_sum"
  V_sum/1 -> V_m/1  "v_sum"
  Pitch_deg/1 -> Th_raw/1  "th_fwd"
  Pitch_deg_rev/1 -> Th_raw/2  "th_rev"
  Deck_up/1 -> Mower_raised/2  "deck_up"
  Drive_on_lo/1 -> Drive_on/1  "Drive_on_lo"
  Drive_on_hi/1 -> Drive_on/2  "Drive_on_hi"
  Released/1 -> Braked/1  "released"
  Impl_id_mask/1 -> Impl_code/1  "impl_id"
  Th_raw/1 -> Th_valid/1  "th_raw"
  Braked/1 -> Rel_age/1(fresh)  "braked"
  R_m/1 -> Ref_d/2, R_m_prev/1  "r_m"
  Th_imu/1 -> Th_valid/3  "th_imu"
  Drive_on/1 -> Trip/3  "drive_on"
  V_m/1 -> Fwd/1, Dir/1, V_abs/1  "v_m"
  Impl_code/1 -> Impl_code_u8/1, Impl_code_s/1  "impl_code"
  V_abs/1 -> V_pred/1, Lag/1  "v"
  R_m_prev/1 -> Ref_d_prev/2  "r_m_prev"
  Dir/1 -> A_d/1, Ref_d/1, Ref_d_prev/1  "dir"
  Rel_age/1(ticks) -> Rel_recent/1  "rel_age"
  Th_valid/1 -> Th_dmx/1  "th"
  Fwd/1 -> Cap_dir/2, Ref_cap_dir/2  "fwd"
  Impl_code_u8/1 -> Impl_other/2, Is_mower/1  "impl_code_u8"
  Th_dmx/1 -> Th_f_taps/1  "th_f"
  Th_dmx/2 -> Th_r_taps/1  "th_r"
  Rel_recent/1 -> Hill_start/1  "rel_recent"
  Zero/1 -> A_pos/2, Dv_used/1  "zero"
  A_d/1 -> A_pos/1  "a_dir"
  Ref_d_prev/1 -> Fall_lim/1  "ref_prev"
  Eps_fall/1 -> Fall_lim/2  "eps_fall"
  Impl_other/1 -> Impl_unknown/1  "impl_other"
  Ref_d/1 -> Falling/1, Ref_still/1, Ref_above/1, Lag/2  "ref"
  Is_mower/1 -> Mower_raised/1  "is_mower"
  Fall_lim/1 -> Falling/2  "fall_lim"
  Lag/1 -> Lag_big/1  "lag"
  A_pos/1 -> Dv_pred/1  "a_pos"
  Impl_unknown/1 -> Row/2  "impl_unknown"
  Ref_still/1 -> Hill_start/2  "ref_still"
  Row_raised_c/1 -> Row_raised/1  "row_raised_c"
  Mower_raised/1 -> Row_raised/2  "mower_raised"
  Th_f_taps/1 -> Th_f_peak/1  "th_f_taps"
  Th_r_taps/1 -> Th_r_peak/1  "th_r_taps"
  Impl_code_s/1 -> Row_raised/3  "impl_code_s"
  Hill_start/1 -> Dv_used/2  "hill_start"
  Dv_pred/1 -> Dv_used/3  "dv_pred"
  Falling/1 -> Decel/1  "falling"
  Th_f_peak/1 -> Th_f_neg/1  "th_f_peak"
  Row_unknown/1 -> Row/1  "row_unknown"
  Th_r_peak/1 -> Th_r_neg/1  "th_r_peak"
  Lag_big/1 -> No_follow/2  "lag_big"
  Row_raised/1 -> Row/3  "row_known"
  Th_f_neg/1 -> Cap_trip_f/2, Cap_ref_f/2  "th_f_neg"
  Th_r_neg/1 -> Cap_trip_r/2, Cap_ref_r/2  "th_r_neg"
  Dv_used/1 -> V_pred/2  "dv_used"
  Row/1 -> Cap_trip_f/1, Cap_ref_r/1, Cap_ref_f/1, Cap_trip_r/1  "row"
  V_pred/1 -> Past_cap/1  "v_pred"
  Cap_trip_f/1 -> Cap_dir/1  "trip_fwd"
  Cap_ref_f/1 -> Ref_cap_dir/1  "ref_cap_fwd"
  Cap_trip_r/1 -> Cap_dir/3  "trip_rev"
  Cap_ref_r/1 -> Ref_cap_dir/3  "ref_cap_rev"
  Cap_dir/1 -> Past_cap/2  "trip_dir"
  Ref_cap_dir/1 -> Ref_above/2  "ref_cap"
  Ref_above/1 -> Cap_pulls/1  "ref_above"
  Past_cap/1 -> Trip/1  "past_cap"
  Cap_pulls/1 -> Decel/2  "cap_pulls"
  Decel/1 -> Steady/1  "decel"
  Steady/1 -> No_follow/1  "steady"
  No_follow/1 -> Trip/2  "no_follow"
  Trip/1 -> cap_trip/1  "cap_trip"

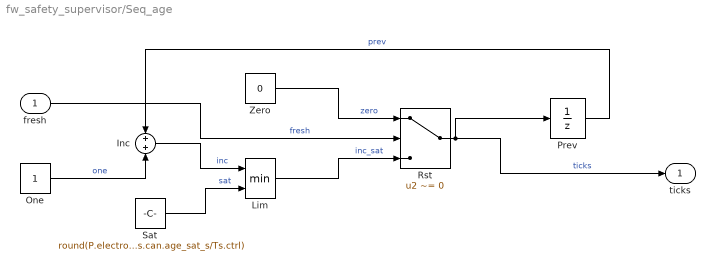
== system fw_safety_supervisor/Seq_age ==
  fresh : Inport
  Inc : Sum  OutDataTypeStr=uint16  SaturateOnIntegerOverflow=on
  Lim : MinMax  Inputs=2
  One : Constant  OutDataTypeStr=uint16  SampleTime=-1
  Prev : UnitDelay  InitialCondition=round(P.electronics.can.age_sat_s/Ts.ctrl)  SampleTime=-1
  Rst : Switch  Criteria=u2 ~= 0  SaturateOnIntegerOverflow=off  InputSameDT=off
  Sat : Constant  Value=round(P.electronics.can.age_sat_s/Ts.ctrl)  OutDataTypeStr=uint16  SampleTime=-1
  Zero : Constant  Value=0  OutDataTypeStr=uint16  SampleTime=-1
  ticks : Outport
  wires:
  fresh/1 -> Rst/2  "fresh"
  One/1 -> Inc/2  "one"
  Inc/1 -> Lim/1  "inc"
  Sat/1 -> Lim/2  "sat"
  Zero/1 -> Rst/1  "zero"
  Lim/1 -> Rst/3  "inc_sat"
  Rst/1 -> ticks/1, Prev/1  "ticks"
  Prev/1 -> Inc/1  "prev"

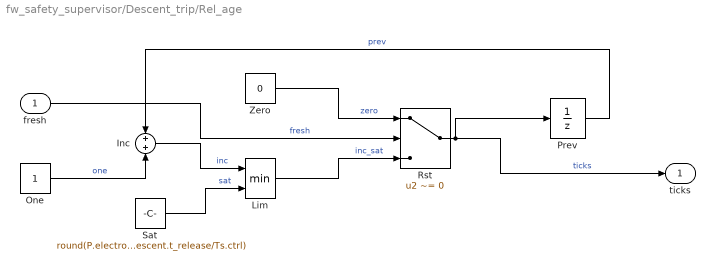
== system fw_safety_supervisor/Descent_trip/Rel_age ==
  fresh : Inport
  Inc : Sum  OutDataTypeStr=uint16  SaturateOnIntegerOverflow=on
  Lim : MinMax  Inputs=2
  One : Constant  OutDataTypeStr=uint16  SampleTime=-1
  Prev : UnitDelay  SampleTime=-1
  Rst : Switch  Criteria=u2 ~= 0  SaturateOnIntegerOverflow=off  InputSameDT=off
  Sat : Constant  Value=round(P.electronics.lim.descent.t_release/Ts.ctrl)  OutDataTypeStr=uint16  SampleTime=-1
  Zero : Constant  Value=0  OutDataTypeStr=uint16  SampleTime=-1
  ticks : Outport
  wires:
  fresh/1 -> Rst/2  "fresh"
  One/1 -> Inc/2  "one"
  Inc/1 -> Lim/1  "inc"
  Sat/1 -> Lim/2  "sat"
  Zero/1 -> Rst/1  "zero"
  Lim/1 -> Rst/3  "inc_sat"
  Rst/1 -> ticks/1, Prev/1  "ticks"
  Prev/1 -> Inc/1  "prev"
